simulink model "Lab2_VM_Auto_Tuning"  (R2026a)
settings: Solver=FixedStepDiscrete  StopTime=Inf  FixedStep=0.02  EnableMultiTasking=on
undefined symbols (not defined in the file or in its folder): Angular, Linear
libraries: robotlib x3, slctrl_autotuning x1, slpidlib x1
settings Model: Creator=The MathWorks, Inc.  LastModifiedBy=juulg
settings OptimizationCC: LifeSpan=Inf
settings HardwareCC: ProdHWDeviceType=Generic->Unspecified (assume 32-bit Generic)  TargetHWDeviceType=Generic->Unspecified (assume 32-bit Generic)  UseEmbeddedCoderFeatures=off
settings SFSimCC: SimTargetLang=C++
settings RTWCC: SystemTargetFile=ert.tlc  HardwareBoard=Robot Operating System (ROS)  Toolchain=Catkin  TargetLang=C++  Description=Embedded Coder
settings ERTTargetCC: RootIOFormat=Structure reference  DynamicArrayContainerType=coder::array  MultiwordLength=2048.0  ERTCustomFileBanners=off  CodeInterfacePackaging=C++ class  SubcomponentCodeInterfacePackaging=C++ class  SupportContinuousTime=on  SupportNonInlinedSFcns=on  SupportVariableSizeSignals=on  ModelStepFunctionPrototypeControlCompliant=off

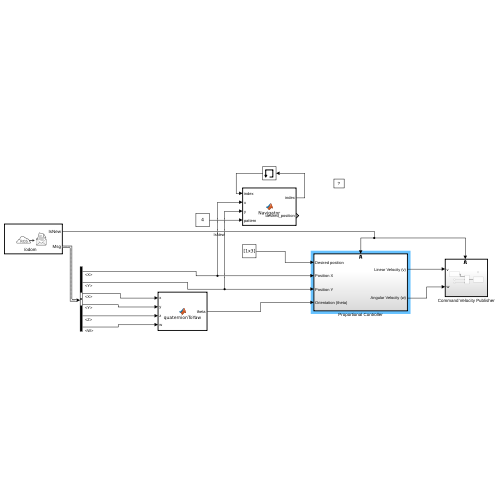
[thumbnail: Simulink's stored preview of the top-level diagram]
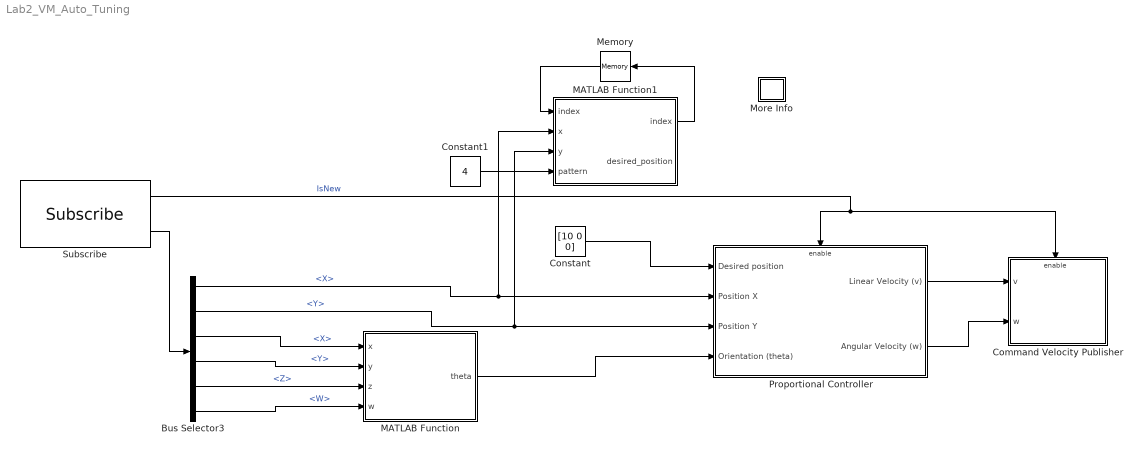
== system Lab2_VM_Auto_Tuning ==
  Bus Selector3 : BusSelector  OutputSignals=Pose.Pose.Position.X,Pose.Pose.Position.Y,Pose.Pose.Orientation.X,Pose.Pose.Orientation.Y,Pose.Pose.Orientation.Z,Pose.Pose.Orientation.W
  Command Velocity Publisher : Subsystem
  Constant : Constant  Value=[10 0 0]  VectorParams1D=off
  Constant1 : Constant  Value=4
  MATLAB Function : MATLAB Function  TreatAsAtomicUnit=on
  MATLAB Function1 : MATLAB Function  TreatAsAtomicUnit=on
  Memory : Memory  InitialCondition=1
  More Info : Subsystem
      settings: OpenFcn=showdemo(bdroot(gcb))
      mask Display: disp('?')
  Proportional Controller : Subsystem
  Subscribe : robotlib/Subscribe  topicSource=Select from ROS network  topic=/odom  messageType=nav_msgs/Odometry  SampleTime=-1  legacyBusStruct=off  messageQueueLength=51
  wires:
  Subscribe/2 -> Bus Selector3/1
  Proportional Controller/1(Linear Velocity (v)) -> Command Velocity Publisher/1(v)
  Subscribe/1 -> Command Velocity Publisher/Enable, Proportional Controller/Enable  "IsNew"
  Bus Selector3/4 -> MATLAB Function/2(y)  "<Y>"
  Proportional Controller/2(Angular Velocity (w)) -> Command Velocity Publisher/2(w)
  Bus Selector3/2 -> MATLAB Function1/3(y), Proportional Controller/3(Position Y)  "<Y>"
  Bus Selector3/1 -> MATLAB Function1/2(x), Proportional Controller/2(Position X)  "<X>"
  MATLAB Function/1(theta) -> Proportional Controller/4(Orientation (theta))
  Bus Selector3/6 -> MATLAB Function/4(w)  "<W>"
  Bus Selector3/5 -> MATLAB Function/3(z)  "<Z>"
  Bus Selector3/3 -> MATLAB Function/1(x)  "<X>"
  MATLAB Function1/1(index) -> Memory/1
  Memory/1 -> MATLAB Function1/1("index ")
  Constant1/1 -> MATLAB Function1/4(pattern)
  Constant/1 -> Proportional Controller/1(Desired position)

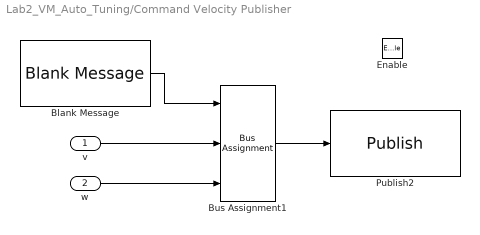
== system Lab2_VM_Auto_Tuning/Command Velocity Publisher ==
  v : Inport
  w : Inport  Port=2
  Enable : EnablePort
  Blank Message : robotlib/Blank Message  messageClass=Message  entityType=geometry_msgs/Twist  messageType=geometry_msgs/Twist  SampleTime=inf  legacyBusStruct=off
  Bus Assignment1 : BusAssignment  DialogController=Simulink.DDGSource_BusAssignment  AssignedSignals=Linear.X,Angular.Z
  Publish2 : robotlib/Publish  topicSource=Select from ROS network  topic=/cmd_vel  messageType=geometry_msgs/Twist  legacyBusStruct=off  messageQueueLength=105
  wires:
  Bus Assignment1/1 -> Publish2/1
  Blank Message/1 -> Bus Assignment1/1
  v/1 -> Bus Assignment1/2
  w/1 -> Bus Assignment1/3

== system Lab2_VM_Auto_Tuning/More Info ==

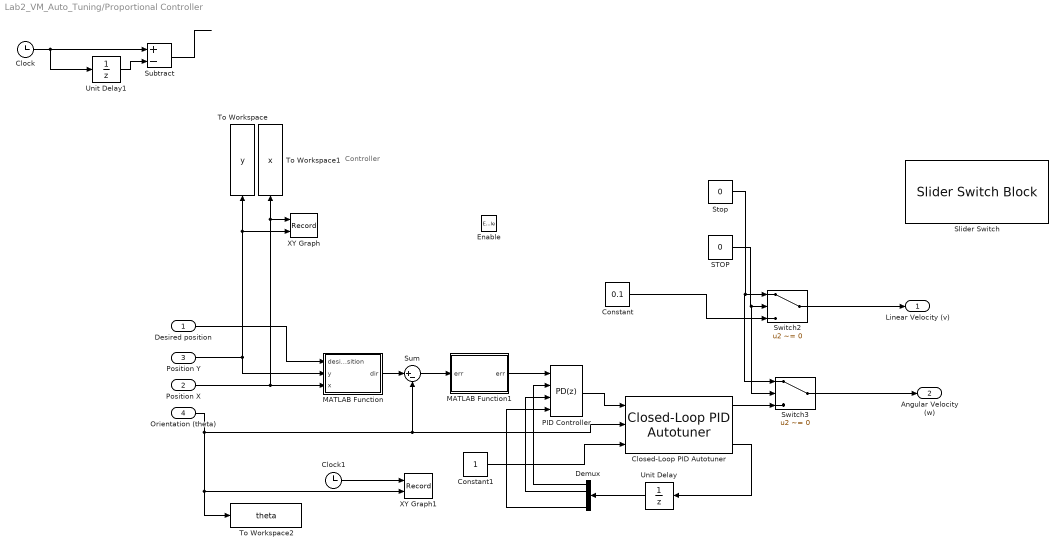
== system Lab2_VM_Auto_Tuning/Proportional Controller ==
  note: Controller
  Desired position : Inport
  Position X : Inport  Port=2
  Position Y : Inport  Port=3
  Orientation (theta) : Inport  Port=4
  Enable : EnablePort
  Clock : Clock
  Clock1 : Clock
  Closed-Loop PID Autotuner : slctrl_autotuning/Closed-Loop PID Autotuner  PIDType=PD  PIDForm=Parallel  TimeDomain=discrete-time  DiscreteTs=0.02  TuningTs=0.2  UseTuningTs=off  IntegratorFormula=Forward Euler  FilterFormula=Forward Euler  ContinuousTs=0.02  Bandwidth=1  UseExternalWC=off  TargetPM=60  UseExternalPM=off  UseExternalAchievedPM=off  ExperimentMode=Superposition  PlantType=Stable  PlantSign=Positive  AmpSine=1  UseExternalAmpSine=off  UseExternalFRD=off  UseExternalU0=off  UseCompanion=off  NotDeployTuningModule=off  UsePLCCoder=off  OutputMode=control action + perturbation  BlockDataType=double  UseExperimentGoodPort=off  UseConnectedPID=on  blockpath=[]  tunedP=0  tunedI=0  tunedD=0  tunedN=100  tunedPM=0  EstimationWindowSize=1  UseExternalTuningParams=off  SingleMultiRateVariant=SingleSamplingRate  NumEstimationPeriods=8  NumSettlingPeriods=2  NumOfPRBSPeriod=1  PRBSSignalOrder=12  ExperimentModeVariant=VariantSuperimposed  OutputChoice=VariantCandD  ConvergenceCalcVariant=ConvSuperpositionPRBSVariant
  Constant : Constant  Value=0.1
  Constant1 : Constant
  Demux : Demux
  MATLAB Function : MATLAB Function  TreatAsAtomicUnit=on
  MATLAB Function1 : MATLAB Function  TreatAsAtomicUnit=on
  PID Controller : slpidlib/PID Controller  Controller=PD  Form=Parallel  TimeDomain=Discrete-time  UseExternalTs=off  SampleTime=-1  IntegratorMethod=Forward Euler  FilterMethod=Forward Euler  ControllerParametersSource=external  P=0.001  I=1  UseKiTs=off  D=0.001  UseExternalDerivativeSource=off  N=100  UseFilter=on  TunerSelectOption=Transfer Function Based (PID Tuner App)  InitialConditionSource=internal  InitialConditionForIntegrator=0  InitialConditionForFilter=0  DifferentiatorICPrevScaledInput=0  ExternalReset=none  TrackingMode=off  Kt=1  LimitOutput=off  SatLimitsSource=internal  UpperSaturationLimit=inf  LowerSaturationLimit=-inf  LinearizeAsGain=on  AntiWindupMode=none  Kb=1  LimitIntegrator=off  UpperIntegratorSaturationLimit=inf  LowerIntegratorSaturationLimit=-inf  POutMin=[]  POutMax=[]  IOutMin=[]  IOutMax=[]  DOutMin=[]  DOutMax=[]  NOutMin=[]  NOutMax=[]  SumOutMin=[]  SumOutMax=[]  SaturationOutMin=[]  SaturationOutMax=[]  PParamMin=[]  PParamMax=[]  IParamMin=[]  IParamMax=[]  DParamMin=[]  DParamMax=[]  NParamMin=[]  NParamMax=[]  KbParamMin=[]  KbParamMax=[]  KtParamMin=[]  KtParamMax=[]  KbOutMin=[]  KbOutMax=[]  KtOutMin=[]  KtOutMax=[]  IntegratorOutMin=[]  IntegratorOutMax=[]  FilterOutMin=[]  FilterOutMax=[]  SumI1OutMin=[]  SumI1OutMax=[]  SumI2OutMin=[]  SumI2OutMax=[]  SumI3OutMin=[]  SumI3OutMax=[]  SumI4OutMin=[]  SumI4OutMax=[]  SumDOutMin=[]  SumDOutMax=[]  DifferentiatorOutMin=[]  DifferentiatorOutMax=[]  FilterDiffOutCoefMin=[]  FilterDiffOutCoefMax=[]  ReciprocalOutMin=[]  ReciprocalOutMax=[]  SumDenOutMin=[]  SumDenOutMax=[]  SumNumOutMin=[]  SumNumOutMax=[]  DivideOutMin=[]  DivideOutMax=[]  UdiffTsProdOutMin=[]  UdiffTsProdOutMax=[]  NTsProdOutMin=[]  NTsProdOutMax=[]  UintegralTsProdOutMin=[]  UintegralTsProdOutMax=[]  UngainTsProdOutMin=[]  UngainTsProdOutMax=[]  ClampingZeroOutDataTypeStr=Inherit: Inherit via back propagation  ClampingZeroOutMin=[]  ClampingZeroOutMax=[]  FilterDenConstantOutDataTypeStr=Inherit: Inherit via back propagation  FilterDenConstantOutMin=[]  FilterDenConstantOutMax=[]  PCopyOutDataTypeStr=Inherit: Inherit via back propagation  PCopyOutMin=[]  PCopyOutMax=[]  NCopyOutDataTypeStr=Inherit: Inherit via back propagation  NCopyOutMin=[]  NCopyOutMax=[]  IntegratorContinuousStateAttributes=''  IntegratorStateMustResolveToSignalObject=off  IntegratorRTWStateStorageClass=Auto  FilterContinuousStateAttributes=''  FilterStateMustResolveToSignalObject=off  FilterRTWStateStorageClass=Auto  ParallelPVariant=ExternalParameters  IdealPVariant=Disabled  IVariant=Disabled  DVariant=ExternalParameters  IntegratorVariant=Disabled  SatVariant=Disabled  AWVariant=Disabled  PCopyVariant=Disabled  TRVariant=Disabled  FdbkBlocksVariant=Forward  IdealPFdbkVariant=Disabled  SatFdbkVariant=Disabled  DerivativeFilterVariant=ForwardEulerFilter  NVariant=ExternalParameters  NCopyVariant=Disabled  FilterICVariant=InternalICsFilter  IntegratorICVariant=Disabled  ExternalResetVariant=Disabled  TRSumVariant=Passthrough  SumFdbkVariant=Disabled  SumVariant=Sum_PD  TsampFilterVariant=InternalTs  TsampNgainVariant=Passthrough  TsampIntegralVariant=Disabled_SignalSpec  ExternalSaturationOutDataTypeStr=Inherit: Same as second input  DerivativeSourceVariant=ErrorSignal  PreIntVariant=InternalPreInt
  "STOP " : Constant  Value=0
  Slider Switch : SliderSwitchBlock
  Stop : Constant  Value=0
  Subtract : Sum  Inputs=+-
  Sum : Sum  Inputs=|+-
  Switch2 : Switch  Criteria=u2 ~= 0  SaturateOnIntegerOverflow=off  InputSameDT=off
  Switch3 : Switch  Criteria=u2 ~= 0  SaturateOnIntegerOverflow=off  InputSameDT=off
  To Workspace : ToWorkspace  VariableName=y  SaveFormat=Timeseries  SampleTime=-1
  To Workspace1 : ToWorkspace  VariableName=x  SaveFormat=Timeseries  SampleTime=-1
  To Workspace2 : ToWorkspace  VariableName=theta  SaveFormat=Timeseries  SampleTime=-1
  Unit Delay : UnitDelay  InitialCondition=[0.01, 0.01, 0, 100]  SampleTime=-1
  Unit Delay1 : UnitDelay  SampleTime=-1
  XY Graph : Record  NumPorts=2.0  FileSettingsInternal="{\"entries\":[{\"content\":{\"excelSettings\":{\"content\":{},\"type\":\"Streamout.ExcelSettings\"},\"parquetSettings\":{\"content\":{},\"type\":\"Streamout.ParquetSettings\"}},\"type\":\"Streamout.FileSettingStorage\",\"uuid\":\"\"}],\"packageUris\":[\"http:\\/\\/schema.mathworks.com\\/mf0\\/streamout_blocks\\/R2020a\"],\"version\":\"1.0\"}"  FrameSettings=[0, 0]  Layout=[1 1]  SignalsInternal="{\"entries\":[{\"content\":{\"signals\":[{\"content\":{\"blockPath\":[],\"dimensions\":[1],\"domain\":\"\",\"lineColor\":\"#a2142f\",\"plots\":[ 1 ],\"port\":1,\"sid\":[\"\"],\"signalID\":1,\"signalName\":\"X\"},\"type\":\"RecordBlkView.Signal\",\"uuid\":\"\"},{\"content\":{\"blockPath\":[],\"dimensions\":[1],\"domain\":\"\",\"lineColor\":\"#139fff\",\"plots\":[ 1 ],\"port\":2,\"sid\":[\"\"],\"signalID\":2,\"signalName\":\"Y\"},\"type\":\"RecordBlkView.Signal\",\"uuid\":\"\"}]},\"type\":\"RecordBlkView.InputSignals\",\"uuid\":\"\"}],\"packageUris\":[\"http:\\/\\/schema.mathworks.com\\/mf0\\/streamout_blocks\\/R2020a\"],\"version\":\"1.0\"}"  VisualizationBindings="{\"xyplotplugin\":{\"info\":[{\"series\":[{\"bindingParametersList\":[{\"parameter\":\"X-Axis\",\"signalID\":1,\"signalName\":\"X\"},{\"parameter\":\"Y-Axis\",\"signalID\":2,\"signalName\":\"Y\"}],\"seriesID\":0}],\"subplotID\":1}]}}"  CompatibilityTag=XY
  XY Graph1 : Record  NumPorts=2.0  FileSettingsInternal="{\"entries\":[{\"content\":{\"excelSettings\":{\"content\":{},\"type\":\"Streamout.ExcelSettings\"},\"parquetSettings\":{\"content\":{},\"type\":\"Streamout.ParquetSettings\"}},\"type\":\"Streamout.FileSettingStorage\",\"uuid\":\"\"}],\"packageUris\":[\"http:\\/\\/schema.mathworks.com\\/mf0\\/streamout_blocks\\/R2020a\"],\"version\":\"1.0\"}"  FrameSettings=[0, 0]  Layout=[1 1]  SignalsInternal="{\"entries\":[{\"content\":{\"signals\":[{\"content\":{\"blockPath\":[],\"dimensions\":[1],\"domain\":\"\",\"lineColor\":\"#a2142f\",\"plots\":[ 1 ],\"port\":1,\"sid\":[\"\"],\"signalID\":1,\"signalName\":\"Clock1\"},\"type\":\"RecordBlkView.Signal\",\"uuid\":\"\"},{\"content\":{\"blockPath\":[],\"dimensions\":[1],\"domain\":\"\",\"lineColor\":\"#139fff\",\"plots\":[ 1 ],\"port\":2,\"sid\":[\"\"],\"signalID\":2,\"signalName\":\"theta\"},\"type\":\"RecordBlkView.Signal\",\"uuid\":\"\"}]},\"type\":\"RecordBlkView.InputSignals\",\"uuid\":\"\"}],\"packageUris\":[\"http:\\/\\/schema.mathworks.com\\/mf0\\/streamout_blocks\\/R2020a\"],\"version\":\"1.0\"}"  VisualizationBindings="{\"xyplotplugin\":{\"info\":[{\"series\":[{\"bindingParametersList\":[{\"parameter\":\"X-Axis\",\"signalID\":1,\"signalName\":\"Clock1\"},{\"parameter\":\"Y-Axis\",\"signalID\":2,\"signalName\":\"theta\"}],\"seriesID\":0}],\"subplotID\":1}]}}"  CompatibilityTag=XY
  Linear Velocity (v) : Outport  VectorParamsAs1DForOutWhenUnconnected=off
  Angular Velocity (w) : Outport  Port=2  VectorParamsAs1DForOutWhenUnconnected=off
  wires:
  Stop/1 -> Switch3/1, Switch2/1
  "STOP "/1 -> Switch3/2, Switch2/2
  Switch2/1 -> Linear Velocity (v)/1
  Switch3/1 -> Angular Velocity (w)/1
  Position X/1 -> MATLAB Function/3(x), To Workspace1/1, XY Graph/1
  Position Y/1 -> MATLAB Function/2(y), To Workspace/1, XY Graph/2
  Constant/1 -> Switch2/3
  Clock/1 -> Unit Delay1/1, Subtract/1
  Unit Delay1/1 -> Subtract/2
  Subtract/1 -> ?
  MATLAB Function/1(dir) -> Sum/1
  Desired position/1 -> MATLAB Function/1(desired_position)
  Orientation (theta)/1 -> Closed-Loop PID Autotuner/2, Sum/2, XY Graph1/2, To Workspace2/1
  Sum/1 -> MATLAB Function1/1("err ")
  MATLAB Function1/1(err) -> PID Controller/1
  Clock1/1 -> XY Graph1/1
  PID Controller/1 -> Closed-Loop PID Autotuner/1
  Closed-Loop PID Autotuner/1 -> Switch3/3
  Constant1/1 -> Closed-Loop PID Autotuner/3
  Closed-Loop PID Autotuner/3 -> Unit Delay/1
  Demux/1 -> PID Controller/2
  Demux/2 -> PID Controller/3
  Demux/4 -> PID Controller/4
  Unit Delay/1 -> Demux/1

== matlab function Lab2_VM_Auto_Tuning/Proportional Controller/MATLAB Function ==
  data: desired_position input; dir output; y input; x input
function dir = Angle(desired_position,y,x)
    position = [x y];
    direction =desired_position(1:2)-position;
    dir = atan2(direction(2),direction(1));
    dir = mod(dir + pi, 2*pi) - pi;
end

== matlab function Lab2_VM_Auto_Tuning/MATLAB Function1 ==
  data: index output; index input; desired_position output; x input; y input; pattern input
function [index,desired_position] = Navigator(index, x,y, pattern)
    square_motion = [0 10; 10 10; 10 0; 0 0];
    j_motion = [
    0 0;
    5.6533 0;
    5.6533 -8.1659;
    3.3501 -9.4221;
    0.8375 -9.2128;
    0 -7.3283
    ];
    i = linspace(0,360,20).';
    sin_motion = [i/9, 10*sin(deg2rad(i))];
    straight_motion=[i,zeros(1, length(i))'];
    % Store paths in a cell array
    patterns = {square_motion, j_motion, sin_motion, straight_motion};

    % Select current path
    current_pattern = patterns{pattern};

    % Get current waypoint
    desired_position = current_pattern(index,:);

    % Check distance to waypoint
    if norm(desired_position(1:2) - [x y]) < 0.12

        index = mod(index, size(current_pattern,1)) + 1;

        % Update desired waypoint
        desired_position = current_pattern(index,:);
    end
end

== matlab function Lab2_VM_Auto_Tuning/MATLAB Function ==
  data: x input; theta output; y input; z input; w input
function theta = quaternionToYaw(x,y,z,w)

    theta = atan2(2*(w*z + x*y), ...
                  1 - 2*(y*y + z*z));

end

== matlab function Lab2_VM_Auto_Tuning/Proportional Controller/MATLAB Function1 ==
  data: err input; err output
function err = wrap(err)
    err = mod(err + pi, 2*pi) - pi;
end
